simulink model "IRMessung2"  (R2026b)
settings: Solver=FixedStepDiscrete  StopTime=inf  FixedStep=0.01  EnableMultiTasking=on
model workspace (MAT data in the model file):
  PAR_FltIr_Fenster_f64 = 9
  PAR_SenIr_Abtast_f64 = Simulink.Parameter
  PAR_SenIr_Abtast_f64.Value = 0.01
  PAR_SenIr_Abtast_f64.Complexity = 'real'
  PAR_SenIr_Abtast_f64.Dimensions = [1 1]
  PAR_SenIr_Abtast_f64.DataType = 'double'
  PAR_SenIr_URef_f32 = Simulink.Parameter
  PAR_SenIr_URef_f32.Value = 5
  PAR_SenIr_URef_f32.Complexity = 'real'
  PAR_SenIr_URef_f32.Dimensions = [1 1]
  PAR_SenIr_URef_f32.DataType = 'single'
libraries: arduinolib x1
settings Model: SILPILModeSetting=veronly
settings SolverCC: AutoInsertRateTranBlk=on
settings OptimizationCC: DifferentSizesBufferReuse=on  EfficientTunableParamExpr=on  EnhancedBackFolding=on  MaxStackSize=64  OptimizationCustomize=off  OptimizeBlockOrder=speed  PassReuseOutputArgsAs=Individual arguments  RemoveInternalMemoryZeroInit=on  RemoveRootLevelIOMemoryZeroInit=on
settings DebuggingCC: ParameterTunabilityLossMsg=error
settings HardwareCC: ProdHWDeviceType=Atmel->AVR  ProdLargestAtomicFloat=None
settings SFSimCC: MATLABDynamicMemAlloc=off
settings RTWCC: BuildConfiguration=Faster Runs  Description=Embedded Coder  HardwareBoard=Arduino Uno  SystemTargetFile=ert.tlc  TLCOptions=-aInlineSetEventsForThisBaseRateFcn=TLC_FALSE -aSuppressMultiTaskScheduler=TLC_FALSE -aRateBasedStepFcn=1  TemplateMakefile=ert_default_tmf  Toolchain=Arduino AVR
settings CodeAppCC: ForceParamTrailComments=on  IgnoreCustomStorageClasses=off  InsertBlockDesc=on  OperatorAnnotations=on  SFDataObjDesc=on  SimulinkDataObjDesc=on
settings ERTTargetCC: CombineSignalStateStructs=on  ExtModeAutomaticAllocSize=off  ExtModeIntrfLevel=Level2 - Open  ExtModeMexFile=ext_xcp  ExtModeStaticAlloc=on  SupportContinuousTime=on  SupportVariableSizeSignals=on

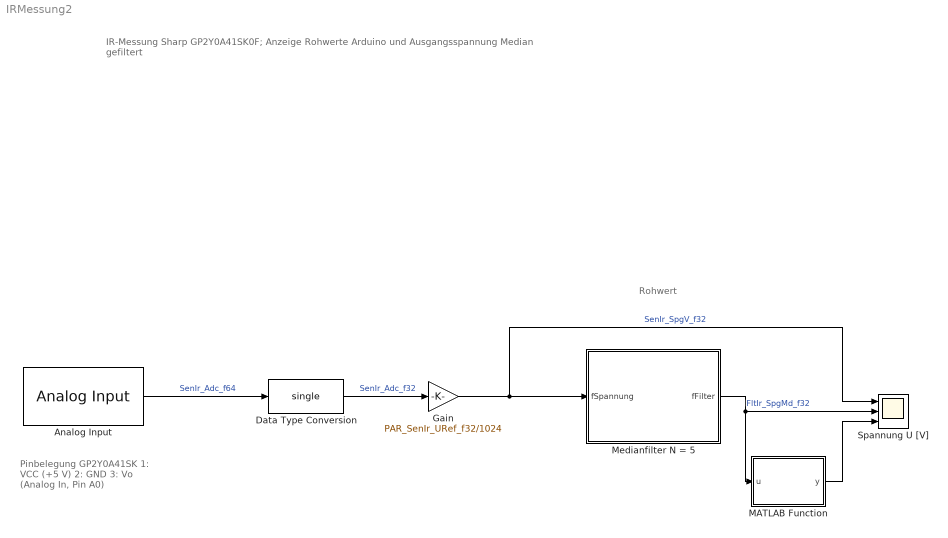
== system IRMessung2 ==
  note: Rohwert
  note: Pinbelegung GP2Y0A41SK
      | 1: VCC (+5 V)
      | 2: GND
      | 3: Vo (Analog In, Pin A0)
  note: IR-Messung Sharp GP2Y0A41SK0F; Anzeige Rohwerte Arduino und Ausgangsspannung Median gefiltert
  Analog Input : arduinolib/Analog Input  pinNumber=0  ReadResultsOnly=off  ConversionTriggerSource=Software  ExternalTriggerType=uint32( 0 )  OutputDataType=uint16  EnableConversionCompleteNotify=off  EnableOuputStatus=off  SampleTime=PAR_SenIr_Abtast_f64  blockPlatform=arduino
  Data Type Conversion : DataTypeConversion  OutDataTypeStr=single  SaturateOnIntegerOverflow=off  RndMeth=Floor
  Gain : Gain  Gain=PAR_SenIr_URef_f32/1024
  MATLAB Function : MATLAB Function  TreatAsAtomicUnit=on
  Medianfilter N = 5 : MATLAB Function  TreatAsAtomicUnit=on
  Spannung U [V] : Scope  NumInputPorts=3
      settings: ActiveDisplayYMinimum=0.017328619956970437  ActiveDisplayYMaximum=12.051073670387268
  wires:
  Analog Input/1 -> Data Type Conversion/1  "SenIr_Adc_f64"
  Data Type Conversion/1 -> Gain/1  "SenIr_Adc_f32"
  Gain/1 -> Medianfilter N = 5/1(fSpannung), Spannung U [V]/1  "SenIr_SpgV_f32"
  Medianfilter N = 5/1(fFilter) -> MATLAB Function/1(u), Spannung U [V]/2  "FltIr_SpgMd_f32"
  MATLAB Function/1(y) -> Spannung U [V]/3

== matlab function IRMessung2/MATLAB Function ==
  data: u input; y output
function y = fcn(u)

y = 32.2029*exp(-0.8604*u);

== matlab function IRMessung2/Medianfilter N = 5 ==
  data: fFilter output; fSpannung input; PAR_FltIr_Fenster_f64 parameter
function fFilter = FiltereMedian(fSpannung, PAR_FltIr_Fenster_f64)
% FiltereMedian: gleitender Median der letzten N Abtastwerte (Aufgabe 2.2.2)
% Eingang   fSpannung             [1x1 single]: Sensorspannung U [V]
% Parameter PAR_FltIr_Fenster_f64 [1x1]: Fensterlaenge N, ungerade, nicht tunebar [-]
% Ausgang   fFilter               [1x1 single]: Median der letzten N Werte [V]
%
% A2.2.1 Fehlerbild (Erwartung aus Datenblatt und Fachwissen, keine Messung):
%   - Einzelne Spannungsspitzen: gepulste IR-LED (ca. 111 mA) belastet die
%     Versorgung; kein Stuetzkondensator im Aufbau -> stochastisch, Filter hilft
%   - Stufen und Wiederholwerte: ADC-Stufe 4,88 mV; Sensor liefert nur ca. alle
%     16,5 ms einen neuen Wert, Abtastung alle 10 ms -> stochastisch, Filter hilft
%   - Nichtlineare Kennlinie, Einfluss von Reflexion, Farbe und Winkel
%     -> systematisch, Filter hilft nicht, Kalibrierung in A2.3
%
% A2.2.2 Parameter: N = 5 (50 ms). Spitzen bis 2 Abtastwerte Dauer werden
%   vollstaendig entfernt (N >= 2 * Dauer + 1); Verzoegerung (N - 1)/2 = 2
%   Abtastwerte = 20 ms. Variation: N = 3 / 5 / 9 -> 10 / 20 / 40 ms.
%
% A2.2.4 Bewertung fuer statische Messungen:
%   Qualitativ: Spitzen verschwinden, Kippen zwischen ADC-Stufen wird
%   geglaettet, Spruenge folgen ohne Ueberschwingen um 20 ms verzoegert.
%   Mittelwert und systematische Abweichung bleiben unveraendert.
%   Quantitativ (Erwartung): Streuungsverhaeltnis s_Filter/s_roh
%   ca. 0,54 fuer N = 5 bei unabhaengigem normalverteiltem Rauschen
%   (Effizienz des Medians fuer n = 5 ca. 0,70); wegen Wiederholwerten
%   (ca. 3 unabhaengige Werte im Fenster) eher ca. 0,67. Mit Spitzen sinkt
%   s_Filter deutlich staerker. Untergrenze: Quantisierungsrauschen
%   U_LSB/sqrt(12) = 1,4 mV.
%   Messung (Platzhalter, je Stufe 5 / 15 / 25 cm, n = ___):
%   s_roh = ___ mV, s_Filter = ___ mV, Verhaeltnis = ___
%   Unsicherheit in cm erst nach A2.3: u_d = u_U / E(d), E = |dU/dd|
persistent afPuffer bStart
N_FENSTER = PAR_FltIr_Fenster_f64;    % Fensterlaenge [-]

if isempty(bStart)
    bStart = false;
    afPuffer = zeros(N_FENSTER,1,'single');  % letzte N Spannungswerte [V]
end

if ~bStart
    afPuffer(:) = fSpannung;          % Start: Puffer mit erstem Wert fuellen, kein Einbruch auf 0 V
    bStart = true;
end

afPuffer = [afPuffer(2:end); fSpannung];   % aeltesten Wert verwerfen, neuen anhaengen
fFilter = median(afPuffer);
end
